simulink subsystem "Load"  (R2024b)
settings: Solver=VariableStepAuto  StartTime=0.0  StopTime=10.0  RelTol=1e-3
libraries: spsSeriesRLCBranchLib x3
settings Model: Creator=User  LastModifiedBy=User

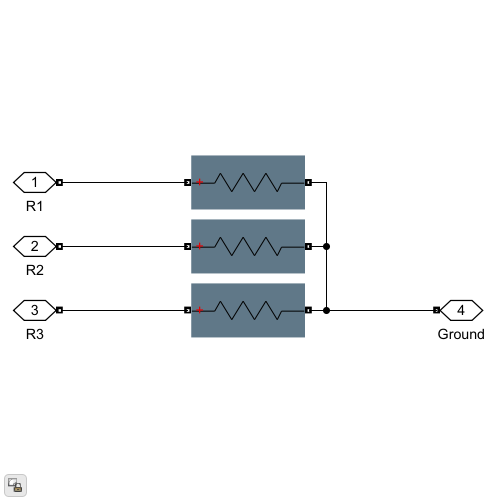
[thumbnail: Simulink's stored preview of the top-level diagram]
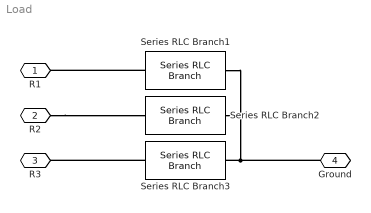
== system Load ==
  Series RLC Branch1 : spsSeriesRLCBranchLib/Series RLC Branch  LConnTagsString=__new0  RConnTagsString=__new0  BranchType=R  Resistance=1  Inductance=1e-3  SetiL0=off  InitialCurrent=0  Capacitance=1e-6  Setx0=off  InitialVoltage=0  Measurements=None
  Series RLC Branch2 : spsSeriesRLCBranchLib/Series RLC Branch  LConnTagsString=__new0  RConnTagsString=__new0  BranchType=R  Resistance=1  Inductance=1e-3  SetiL0=off  InitialCurrent=0  Capacitance=1e-6  Setx0=off  InitialVoltage=0  Measurements=None
  Series RLC Branch3 : spsSeriesRLCBranchLib/Series RLC Branch  LConnTagsString=__new0  RConnTagsString=__new0  BranchType=R  Resistance=1  Inductance=1e-3  SetiL0=off  InitialCurrent=0  Capacitance=1e-6  Setx0=off  InitialVoltage=0  Measurements=None
  R1 : PMIOPort  Side=Left
  R2 : PMIOPort  Port=2  Side=Left
  R3 : PMIOPort  Port=3  Side=Left
  Ground : PMIOPort  Port=4  Side=Right
  connections:
  Series RLC Branch1/RConn1 -- Series RLC Branch3/RConn1 -- Ground/RConn1 -- Series RLC Branch2/RConn1
  Series RLC Branch3/LConn1 -- R3/RConn1
  R2/RConn1 -- Series RLC Branch2/LConn1
  Series RLC Branch1/LConn1 -- R1/RConn1
